simulink model "flight_simulation_6dof"  (R2025b)
settings: Solver=ode4  StartTime=0.0  StopTime=8.6  FixedStep=1/1000  RelTol=1e-3  AbsTol=1e-3  EnableMultiTasking=on
undefined symbols (not defined in the file): X, Y, Z
libraries: nesl_utility x122, sm_lib x98, simulink_extras x48, aerolibatmos2 x4, sharedtransform x4
(part 2 of 6)

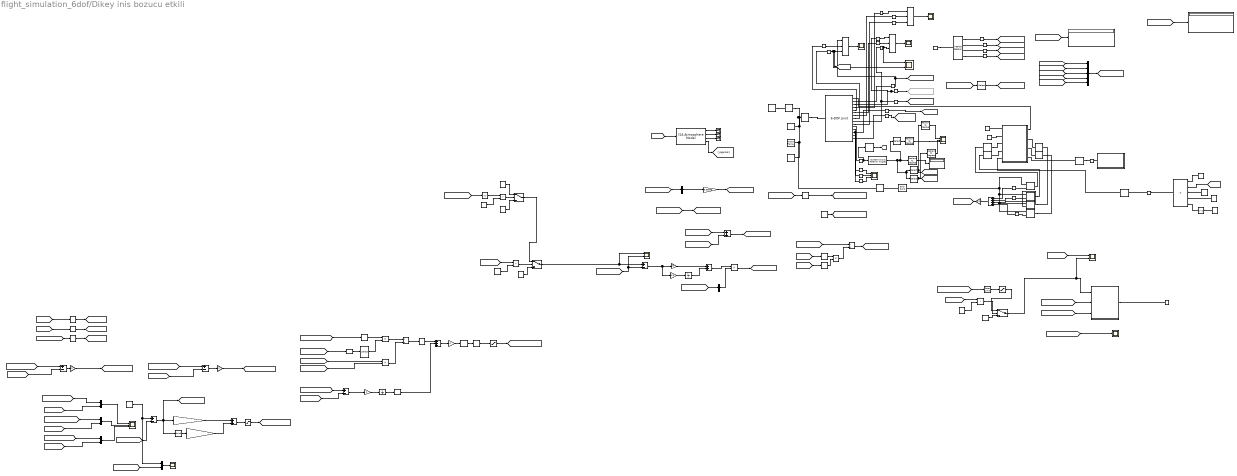
== system flight_simulation_6dof/Dikey inis bozucu etkili ==
  note: 0 itki [N]
  note: Integral Corrector
  note: Ang Velocity to Ang Accel Command
  note: Dynamic Inversion
  note: Ang Velocity to Ang Accel Command
  note: Z Axis
  note: zemine 0.001 metre kala itkiyi 0 yap
  note: Yere 6 metre kala
  note: 6. metreden sonra hizi su olcak
  note: F=1/2 ​ρ.C D. ​A.V rel ​^2
  6-DOF Joint : sm_lib/Joints/6-DOF Joint  JointMode=Normal  CompositeWrenchDir=FollowerOnBase  CompositeWrenchFrame=BaseFrame  SenseConstraintForce=off  SenseConstraintTorque=off  SenseTotalForce=off  SenseTotalTorque=off  PxPositionTargetSpecify=off  PxPositionTargetPriority=High  PxPositionTargetValue=15  PxPositionTargetValueUnits=m  PxVelocityTargetSpecify=off  PxVelocityTargetPriority=High  PxVelocityTargetValue=0  PxVelocityTargetValueUnits=m/s  PxEquilibriumPosition=0  PxEquilibriumPositionUnits=m  PxSpringStiffness=0  PxSpringStiffnessUnits=N/m  PxDampingCoefficient=0  PxDampingCoefficientUnits=N/(m/s)  PxLowerLimitSpecify=off  PxLowerLimitBound=-1  PxLowerLimitBoundUnits=m  PxLowerLimitStiffness=1e6  PxLowerLimitStiffnessUnits=N/m  PxLowerLimitDamping=1e3  PxLowerLimitDampingUnits=N/(m/s)  PxLowerLimitTransitionRegionWidth=1e-4  PxLowerLimitTransitionRegionWidthUnits=m  PxUpperLimitSpecify=off  PxUpperLimitBound=1  PxUpperLimitBoundUnits=m  PxUpperLimitStiffness=1e6  PxUpperLimitStiffnessUnits=N/m  PxUpperLimitDamping=1e3  PxUpperLimitDampingUnits=N/(m/s)  PxUpperLimitTransitionRegionWidth=1e-4  PxUpperLimitTransitionRegionWidthUnits=m  PxTorqueActuationMode=NoTorque  PxMotionActuationMode=ComputedMotion  PxSensePosition=on  PxSenseVelocity=on  PxSenseAcceleration=on  PxSenseTorqueForce=off  PxSenseLowerLimitTorqueForce=off  PxSenseUpperLimitTorqueForce=off  PyPositionTargetSpecify=on  PyPositionTargetPriority=High  PyPositionTargetValue=0  PyPositionTargetValueUnits=m  PyVelocityTargetSpecify=off  PyVelocityTargetPriority=High  PyVelocityTargetValue=0  PyVelocityTargetValueUnits=m/s  PyEquilibriumPosition=0  PyEquilibriumPositionUnits=m  PySpringStiffness=0  PySpringStiffnessUnits=N/m  PyDampingCoefficient=0  PyDampingCoefficientUnits=N/(m/s)  PyLowerLimitSpecify=off  PyLowerLimitBound=-1  PyLowerLimitBoundUnits=m  PyLowerLimitStiffness=1e6  PyLowerLimitStiffnessUnits=N/m  PyLowerLimitDamping=1e3  PyLowerLimitDampingUnits=N/(m/s)  PyLowerLimitTransitionRegionWidth=1e-4  PyLowerLimitTransitionRegionWidthUnits=m  PyUpperLimitSpecify=off  PyUpperLimitBound=1  PyUpperLimitBoundUnits=m  PyUpperLimitStiffness=1e6  PyUpperLimitStiffnessUnits=N/m  PyUpperLimitDamping=1e3  PyUpperLimitDampingUnits=N/(m/s)  PyUpperLimitTransitionRegionWidth=1e-4  PyUpperLimitTransitionRegionWidthUnits=m  PyTorqueActuationMode=NoTorque  PyMotionActuationMode=ComputedMotion  PySensePosition=on  PySenseVelocity=on  PySenseAcceleration=on  PySenseTorqueForce=off  PySenseLowerLimitTorqueForce=off  PySenseUpperLimitTorqueForce=off  PzPositionTargetSpecify=on  PzPositionTargetPriority=High  PzPositionTargetValue=10  PzPositionTargetValueUnits=m  PzVelocityTargetSpecify=off  PzVelocityTargetPriority=High  PzVelocityTargetValue=0  PzVelocityTargetValueUnits=m/s  PzEquilibriumPosition=0  PzEquilibriumPositionUnits=m  PzSpringStiffness=0  PzSpringStiffnessUnits=N/m  PzDampingCoefficient=0  PzDampingCoefficientUnits=N/(m/s)  PzLowerLimitSpecify=off  PzLowerLimitBound=-1  PzLowerLimitBoundUnits=m  PzLowerLimitStiffness=1e6  PzLowerLimitStiffnessUnits=N/m  PzLowerLimitDamping=1e3  PzLowerLimitDampingUnits=N/(m/s)  PzLowerLimitTransitionRegionWidth=1e-4  PzLowerLimitTransitionRegionWidthUnits=m  PzUpperLimitSpecify=off  PzUpperLimitBound=1  PzUpperLimitBoundUnits=m  PzUpperLimitStiffness=1e6  PzUpperLimitStiffnessUnits=N/m  PzUpperLimitDamping=1e3  PzUpperLimitDampingUnits=N/(m/s)  PzUpperLimitTransitionRegionWidth=1e-4  PzUpperLimitTransitionRegionWidthUnits=m  PzTorqueActuationMode=NoTorque  PzMotionActuationMode=ComputedMotion  PzSensePosition=on  PzSenseVelocity=on  PzSenseAcceleration=on  PzSenseTorqueForce=off  PzSenseLowerLimitTorqueForce=off  PzSenseUpperLimitTorqueForce=off  SphPositionTargetSpecify=on  SphPositionTargetPriority=High  SphPositionTargetRotationMethod=StandardAxis  SphPositionTargetFollAlignAxisA=+X  SphPositionTargetBaseAlignAxisA=+Y  SphPositionTargetFollAlignAxisB=+Y  SphPositionTargetBaseAlignAxisB=+Z  SphPositionTargetRotationStandardAxis=+Y  SphPositionTargetRotationAngle=15  SphPositionTargetRotationAngleUnits=deg  SphPositionTargetRotationArbitraryAxis=[1 1 0]  SphPositionTargetRotationSequenceAxes=FollowerAxes  SphPositionTargetRotationSequence=XYX  SphPositionTargetRotationSequenceAngles=[0 0 0]  SphPositionTargetRotationSequenceAnglesUnits=deg  SphPositionTargetRotationMatrix=[1 0 0;0 1 0;0 0 1]  SphPositionTargetQuaternion=[1 0 0 0]  SphVelocityTargetSpecify=off  SphVelocityTargetPriority=High  SphVelocityTargetValue=[0 0 0]  SphVelocityTargetValueUnits=deg/s  SphVelocityTargetInFollowerFrame=on  SphEqPosRotationMethod=None  SphEqPosFollAlignAxisA=+X  SphEqPosBaseAlignAxisA=+Y  SphEqPosFollAlignAxisB=+Y  SphEqPosBaseAlignAxisB=+Z  SphEqPosRotationStandardAxis=+Z  SphEqPosRotationAngle=0  SphEqPosRotationAngleUnits=deg  SphEqPosRotationArbitraryAxis=[0 0 1]  SphEqPosRotationSequenceAxes=FollowerAxes  SphEqPosRotationSequence=XYX  SphEqPosRotationSequenceAngles=[0 0 0]  SphEqPosRotationSequenceAnglesUnits=deg  SphEqPosRotationMatrix=[1 0 0;0 1 0;0 0 1]  SphEqPosQuaternion=[1 0 0 0]  SphSpringStiffness=0  SphSpringStiffnessUnits=N*m/deg  SphDampingCoefficient=0  SphDampingCoefficientUnits=N*m/(deg/s)  SphLowerLimitSpecify=off  SphLowerLimitBound=15  SphLowerLimitBoundUnits=deg  SphLowerLimitStiffness=1e4  SphLowerLimitStiffnessUnits=N*m/deg  SphLowerLimitDamping=10  SphLowerLimitDampingUnits=N*m/(deg/s)  SphLowerLimitTransitionRegionWidth=0.1  SphLowerLimitTransitionRegionWidthUnits=deg  SphUpperLimitSpecify=off  SphUpperLimitBound=45  SphUpperLimitBoundUnits=deg  SphUpperLimitStiffness=1e4  SphUpperLimitStiffnessUnits=N*m/deg  SphUpperLimitDamping=10  SphUpperLimitDampingUnits=N*m/(deg/s)  SphUpperLimitTransitionRegionWidth=0.1  SphUpperLimitTransitionRegionWidthUnits=deg  SphTorqueActuationMode=NoTorque  SphActuateTorqueX=off  SphActuateTorqueY=off  SphActuateTorqueZ=off  SphActuateTorque=off  SphActuationFrame=BaseFrame  SphSensePosition=on  SphSenseVelocityX=on  SphSenseVelocityY=on  SphSenseVelocityZ=on  SphSenseVelocity=off  SphSenseAccelerationX=off  SphSenseAccelerationY=on  SphSenseAccelerationZ=off  SphSenseAcceleration=off  SphSenseLowerLimitTorqueMag=off  SphSenseUpperLimitTorqueMag=off  SphSensingFrame=BaseFrame
  Abs : Abs  SaturateOnIntegerOverflow=off
  Add : Sum
  Add{1..3,5..6} (5 alike) : Sum  Inputs=+-
  Add4 : Sum  Inputs=3
  Add7 : Sum
  Add8 : Sum  Inputs=4
  Add9 : Sum
  Alan : Constant  Value=0.25
  Asin1 : Trigonometry  Operator=asin
  Bus Creator : BusCreator  Inputs=5
  Bus Selector : BusSelector  OutputSignals=mass_kg
  Bus Selector1 : BusSelector  OutputSignals=mass_kg
  CD​≈1 : Constant
  Connection Label16 : ConnectionLabel  Label=FN1
  Connection Label17 : ConnectionLabel  Label=FN1
  Connection Label34 : ConnectionLabel  Label=Nozzle_Frame
  Connection Label35 : ConnectionLabel  Label=Nozzle_Frame
  Constant : Constant  Value=0
  Constant1 : Constant
  Constant2 : Constant  Value=6
  Constant4 : Constant  Value=1/2
  Constant5 : Constant  Value=0
  Constant6 : Constant  Value=-0.08
  Constant7 : Constant  Value=0.001
  Constant8 : Constant  Value=0
  Cos : Trigonometry  Operator=cos
  Cos1 : Trigonometry  Operator=cos
  Degrees to Radians1 : simulink_extras/Transformations/Degrees to Radians
  Degrees to Radians2 : simulink_extras/Transformations/Degrees to Radians
  Delay : Delay  DelayLength=1
  Delay1 : Delay  DelayLength=1  InitialCondition=25000*10
  Derivative : Derivative
  Display : Display
  Display1 : Display
  Display2 : Display
  Divide : Product  Inputs=*/
  Divide2 : Product  Inputs=*/
  External Force and Torque : sm_lib/Forces and Torques/External Force and Torque  EnableForceX=on  EnableForceY=off  EnableForceZ=off  EnableForce=off  ForceResolutionFrame=AttachedFrame  EnableTorqueX=off  EnableTorqueY=off  EnableTorqueZ=off  EnableTorque=off  TorqueResolutionFrame=AttachedFrame
  Floor : sm_lib/Body Elements/Brick Solid  BrickDimensions=[30 30 2]  BrickDimensionsUnits=m  ExportEntireGeometry=on  InertiaType=CalculateFromGeometry  BasedOnType=Density  Density=0  DensityUnits=kg/m^3  Mass=1  MassUnits=kg  CenterOfMass=[0 0 0]  CenterOfMassUnits=m  MomentsOfInertia=[1 1 1]  MomentsOfInertiaUnits=kg*m^2  ProductsOfInertia=[0 0 0]  ProductsOfInertiaUnits=kg*m^2  GraphicType=FromGeometry  MarkerShape=Sphere  MarkerSize=10  GraphicVisPropType=SimpleVisualProperties  GraphicDiffuseColor=[0.4 0.8 0.0]  GraphicOpacity=1  GraphicSpecularColor=[0.5 0.5 0.5 1.0]  GraphicAmbientColor=[0.15 0.15 0.15 1.0]  GraphicEmissiveColor=[0.0 0.0 0.0 1.0]  GraphicShininess=75  DoExposeReferenceFrame=on  SerializedFrames=<Frames/>
  Gain : Gain  Gain=9.80665
  Gain1 : Gain  Gain=1/4
  Gain2 : Gain  Gain=3
  Gain3 : Gain  Gain=0.263030697386858*5
  Gain4 : Gain
  Gain5 : Gain  Gain=2
  Gain6 : Gain  Gain=-1
  Gain7 : Gain  Gain=2
  Gain8 : Gain  Gain=1.772424617277137*2
  Gain9 : Gain  Gain=0.5
  Goto26 : Goto  Commented=on  GotoTag=x_dot_current_m_s
  Graphic : sm_lib/Body Elements/Graphic  GraphicType=Marker  MarkerShape=Cube  MarkerSize=10  GraphicVisPropType=SimpleVisualProperties  GraphicDiffuseColor=[0.5 0.5 0.5]  GraphicOpacity=1  GraphicSpecularColor=[0.5 0.5 0.5 1.0]  GraphicAmbientColor=[0.15 0.15 0.15 1.0]  GraphicEmissiveColor=[0.0 0.0 0.0 1.0]  GraphicShininess=75
  GreaterThan : RelationalOperator  Operator=>  OutDataTypeStr=boolean  RndMeth=Simplest  InputSameDT=off
  GreaterThan1 : RelationalOperator  Operator=>  OutDataTypeStr=boolean  RndMeth=Simplest  InputSameDT=off
  GreaterThan3 : RelationalOperator  Operator=>  OutDataTypeStr=boolean  RndMeth=Simplest  InputSameDT=off
  ISA Atmosphere Model : aerolibatmos2/ISA Atmosphere Model  useExtended=off  action=None  custom=off  viscosityOut=off  g=9.80665  gamma=1.4  R=287.0531  L=0.0065  h_trop=11000  h_strat=20000  rho0=1.225  P0=101325  T0=288.15  h0=0  S=110.4  Tref=273.15  muref=1.716e-5
  Inertia Sensor : sm_lib/Body Elements/Inertia Sensor  SensorExtent=Mechanism  SpanWeldJoints=off  ExcludeGroundedBodies=off  MeasurementFrame=Attached  SenseMass=on  SenseCenterOfMass=on  SenseInertiaMatrix=on  SenseCenteredInertiaMatrix=on  SensePrincipalInertiaMatrix=off  SenseRotationMatrix=off  GraphicType=PrincipalInertiaFrame  PrincipalInertiaFrameSize=20  GraphicVisPropType=SimpleVisualProperties  GraphicDiffuseColor=[0.5 0.5 0.5]  GraphicOpacity=1  GraphicSpecularColor=[0.5 0.5 0.5 1.0]  GraphicAmbientColor=[0.15 0.15 0.15 1.0]  GraphicEmissiveColor=[0.0 0.0 0.0 1.0]  GraphicShininess=75
  Integrator : Integrator  LimitOutput=on  UpperSaturationLimit=10  LowerSaturationLimit=-10
  Integrator1 : Integrator  LimitOutput=on  UpperSaturationLimit=5000*10  LowerSaturationLimit=-5000*10
  MassModel1 : Subsystem
  Mechanism Configuration : sm_lib/Utilities/Mechanism Configuration  UniformGravity=Constant  GravityVector=[0 0 -9.80665]  GravityVectorUnits=m/s^2  LinearizationDelta=0.001  JointModeTransitionNonlinearIterations=2
  Mux{,1..3} (4 alike) : Mux  Inputs=2
  Mux4 : Mux  Inputs=3
  Mux5 : Mux  Inputs=3
  Mux6 : Mux  Inputs=3
  PS-Simulink Converter{,1..24} (25 alike) : nesl_utility/PS-Simulink Converter  PhysicalDomain=network_engine_domain  SubClassName=ps_output  LeftPortType=input  RightPortType=output  PseudoPeriodic=off  Frequencies=[]  VectorFormat=inherit  Unit=inherit  AffineConversion=off
  Product{,1,4..5} (4 alike) : Product
  Product2 : Product  Inputs=5
  Quaternions to Direction Cosine Matrix : Quat2Dcm
  Quaternions to Rotation Angles : sharedtransform/Quaternions to Rotation Angles  rotationOrder=ZYX  aMode=aMode
  Radians to Degrees{,1..4,7..9} (8 alike) : simulink_extras/Transformations/Radians to Degrees
  Rate Limiter : RateLimiter  RisingSlewLimit=500/0.2  FallingSlewLimit=-500/0.2  SampleTimeMode=inherited
  Reshape1 : Reshape
  Rigid Transform : sm_lib/Frames and Transforms/Rigid Transform  RotationMethod=None  FollAlignAxisA=+X  BaseAlignAxisA=+Y  FollAlignAxisB=+Y  BaseAlignAxisB=+Z  RotationStandardAxis=+Z  RotationAngle=0  RotationAngleUnits=deg  RotationArbitraryAxis=[0 0 1]  RotationSequenceAxes=FollowerAxes  RotationSequence=XYX  RotationSequenceAngles=[0 0 0]  RotationSequenceAnglesUnits=deg  RotationMatrix=[1 0 0;0 1 0;0 0 1]  Quaternion=[1 0 0 0]  TranslationMethod=Cartesian  TranslationCartesianOffset=[0 0 0]  TranslationCartesianOffsetUnits=m  TranslationStandardAxis=+Z  TranslationStandardOffset=0  TranslationStandardOffsetUnits=m  TranslationROffset=0  TranslationROffsetUnits=m  TranslationThetaOffset=0  TranslationThetaOffsetUnits=deg  TranslationZOffset=0  TranslationZOffsetUnits=m
  Rigid Transform1 : sm_lib/Frames and Transforms/Rigid Transform  RotationMethod=None  FollAlignAxisA=+X  BaseAlignAxisA=+Y  FollAlignAxisB=+Y  BaseAlignAxisB=+Z  RotationStandardAxis=+Z  RotationAngle=0  RotationAngleUnits=deg  RotationArbitraryAxis=[0 0 1]  RotationSequenceAxes=FollowerAxes  RotationSequence=XYX  RotationSequenceAngles=[0 0 0]  RotationSequenceAnglesUnits=deg  RotationMatrix=[1 0 0;0 1 0;0 0 1]  Quaternion=[1 0 0 0]  TranslationMethod=Cartesian  TranslationCartesianOffset=[0 0 -1.82]  TranslationCartesianOffsetUnits=m  TranslationStandardAxis=+Z  TranslationStandardOffset=0  TranslationStandardOffsetUnits=m  TranslationROffset=0  TranslationROffsetUnits=m  TranslationThetaOffset=0  TranslationThetaOffsetUnits=deg  TranslationZOffset=0  TranslationZOffsetUnits=m
  Rigid Transform2 : sm_lib/Frames and Transforms/Rigid Transform  RotationMethod=None  FollAlignAxisA=+X  BaseAlignAxisA=+Y  FollAlignAxisB=+Y  BaseAlignAxisB=+Z  RotationStandardAxis=+Z  RotationAngle=0  RotationAngleUnits=deg  RotationArbitraryAxis=[0 0 1]  RotationSequenceAxes=FollowerAxes  RotationSequence=XYX  RotationSequenceAngles=[0 0 0]  RotationSequenceAnglesUnits=deg  RotationMatrix=[1 0 0;0 1 0;0 0 1]  Quaternion=[1 0 0 0]  TranslationMethod=Cartesian  TranslationCartesianOffset=[0 0 -1.82]  TranslationCartesianOffsetUnits=m  TranslationStandardAxis=+Z  TranslationStandardOffset=0  TranslationStandardOffsetUnits=m  TranslationROffset=0  TranslationROffsetUnits=m  TranslationThetaOffset=0  TranslationThetaOffsetUnits=deg  TranslationZOffset=0  TranslationZOffsetUnits=m
  Saturation : Saturate  UpperLimit=60  LowerLimit=-60
  Saturation1 : Saturate  UpperLimit=20  LowerLimit=-20
  Saturation2 : Saturate  UpperLimit=500/0.2  LowerLimit=0
  Scope : Scope  NumInputPorts=2
      settings: ActiveDisplayYMinimum=-1.625829118727711  ActiveDisplayYMaximum=0.25053784432938375
  Scope1 : Scope  NumInputPorts=3
      settings: ActiveDisplayYMinimum=-19.808742904399047  ActiveDisplayYMaximum=34.576797333379531
  Scope10 : Scope  NumInputPorts=2
      settings: ActiveDisplayYMinimum=-107.28824489550837  ActiveDisplayYMaximum=965.56718541932582  DataLoggingVariableName=ScopeData9
  Scope11 : Scope  NumInputPorts=3
      settings: ActiveDisplayYMinimum=-22.793707101323157  ActiveDisplayYMaximum=10.917952452796278  DataLoggingVariableName=ScopeData12
  Scope{2,5..7,9} (5 alike) : Scope
      Scope2 settings: ActiveDisplayYMinimum=-1  ActiveDisplayYMaximum=1  DataLoggingVariableName=ScopeData2
      Scope5 settings: ActiveDisplayYMinimum=-11.092753948931176  ActiveDisplayYMaximum=5.4980270582822843  DataLoggingVariableName=ScopeData3
      Scope6 settings: ActiveDisplayYMinimum=-2.6747294131347727  ActiveDisplayYMaximum=11.408303268126085  DataLoggingVariableName=ScopeData4
      Scope7 settings: ActiveDisplayYMinimum=-50.120004759868806  ActiveDisplayYMaximum=49.994550495676052  DataLoggingVariableName=ScopeData5
      Scope9 settings: ActiveDisplayYMinimum=-1  ActiveDisplayYMaximum=1  DataLoggingVariableName=ScopeData8
  Scope4 : Scope  NumInputPorts=2
      settings: ActiveDisplayYMinimum=-9.5328876838367336  ActiveDisplayYMaximum=0.53135333799624407  DataLoggingVariableName=ScopeData7
  Scope8 : Scope  NumInputPorts=3
      settings: ActiveDisplayYMinimum=-25.077488901630971  ActiveDisplayYMaximum=26.517066183158931  DataLoggingVariableName=ScopeData10
  Selector : Selector  InputPortWidth=3  IndexOptions=Index vector (dialog)  Indices=2  OutputSizes=1
  Selector1 : Selector  InputPortWidth=3  IndexOptions=Index vector (dialog)  Indices=3  OutputSizes=1
  Selector2 : Selector  InputPortWidth=3  IndexOptions=Index vector (dialog)  Indices=3  OutputSizes=1
  Selector3 : Selector  InputPortWidth=3  IndexOptions=Index vector (dialog)  Indices=1  OutputSizes=1
  Selector4 : Selector  InputPortWidth=9  IndexOptions=Index vector (dialog)  Indices=5  OutputSizes=1
  Simulink-PS Converter : nesl_utility/Simulink-PS Converter  PhysicalDomain=network_engine_domain  SubClassName=ps_input  LeftPortType=input  RightPortType=output  PseudoPeriodic=off  Frequencies=[]  NoiseDistribution=none  NoiseParameters=[]  Unit=1  AffineConversion=off  FilteringAndDerivatives=provide  SimscapeFilterOrder=1  InputFilterTimeConstant=0.001  UdotUserProvided=0
  Simulink-PS Converter2 : nesl_utility/Simulink-PS Converter  PhysicalDomain=network_engine_domain  SubClassName=ps_input  LeftPortType=input  RightPortType=output  PseudoPeriodic=off  Frequencies=[]  NoiseDistribution=none  NoiseParameters=[]  Unit=1  AffineConversion=off  FilteringAndDerivatives=provide  SimscapeFilterOrder=1  InputFilterTimeConstant=0.001  UdotUserProvided=0
  Solver Configuration : nesl_utility/Solver Configuration  PhysicalDomain=network_engine_domain  SubClassName=solver  LeftPortType=input  RightPortType=generic  Tones=[]  Harmonics=[]  SimulateNoise=off  Profile=off  UseLocalSampling=off  EnableSwitchedLinearOptims=on  FrequencyDomain=off  UseCCode=off  RelTol=0.001  AbsTol=1e-06  MinStep=1e-09  ToWorkspace=off  RevertToSquareIcSolve=off  NumHomotopyIterations=100  PhasorMode=off  PhasorModeNumHarmonics=1  ConsistencySolver=NEWTON_XTOL_AFTER_FTOL  IndexReductionMethod=DerivativeReplacement  DoDC=off  ResidualTolerance=1e-09  ConsistencyTolSource=GLOBAL  ConsistencyAbsTol=0.001  ConsistencyRelTol=0.001  ConsistencyTolFactor=0.001  UseLocalSolver=off  LocalSolverChoice=NE_BACKWARD_EULER_ADVANCER  ResolveIndetEquations=on  FunctionEvalNumThread=1  LocalSolverSampleTime=0.001  DoFixedCost=off  MaxNonlinIter=3  MaxModeIter=2  ComputeImpulses=off  ImpulseIterations=2  LinearAlgebra=Sparse  LinearAlgebraNumThread=0  EquationFormulation=NE_TIME_EF  DelaysMemoryBudget=1024  AutomaticFiltering=on  FilteringTimeConstant=0.001  PartitionStorageMethod=AS_NEEDED  PartitionMemoryBudget=1024  PartitionMethod=FAST  MultibodyUseLocalSolver=off  MultibodyLocalSolverChoice=ODE1  MultibodyLocalSolverSampleTime=0.001
  Spatial Contact Force{,1..3} (4 alike) : sm_lib/Forces and Torques/Spatial Contact Force  SenseSeparationDistance=on  NormalForceType=SmoothSpringDamper  NormalStiffness=3e4  NormalStiffnessUnits=N/m  NormalDamping=8e2  NormalDampingUnits=N/(m/s)  NormalTransitionRegionWidth=1e-3  NormalTransitionRegionWidthUnits=m  FrictionType=SmoothStickSlip  CoefficientOfStaticFriction=0.5  CoefficientOfDynamicFriction=0.3  FrictionalCriticalVelocity=1e-3  FrictionalCriticalVelocityUnits=m/s  SenseContactSignal=off  SensePenetrationDepth=off  SenseNormalVelocity=off  SenseTangentialVelocity=off  SensingForceTorqueDirection=BaseOnFollower  SensingForceTorqueResolutionFrame=ContactFrame  SenseNormalForce=off  SenseNormalForceMagnitude=off  SenseNormalTorque=off  SenseFrictionalForce=off  SenseFrictionalForceMagnitude=off  SenseFrictionalTorque=off  SenseTotalForce=off  SenseTotalTorque=off  SenseContactBaseRotation=off  SenseContactBaseTranslation=off  SenseContactFollowerRotation=off  SenseContactFollowerTranslation=off  ZeroCrossDetectContactStartAndEnd=off
  Spherical Solid{,1..3} (4 alike) : sm_lib/Body Elements/Spherical Solid  SphereRadius=0.01  SphereRadiusUnits=m  ExportEntireGeometry=on  InertiaType=CalculateFromGeometry  BasedOnType=Density  Density=0  DensityUnits=kg/m^3  Mass=1  MassUnits=kg  CenterOfMass=[0 0 0]  CenterOfMassUnits=m  MomentsOfInertia=[1 1 1]  MomentsOfInertiaUnits=kg*m^2  ProductsOfInertia=[0 0 0]  ProductsOfInertiaUnits=kg*m^2  GraphicType=FromGeometry  MarkerShape=Sphere  MarkerSize=10  GraphicVisPropType=SimpleVisualProperties  GraphicDiffuseColor=[0.502 0 0]  GraphicOpacity=1  GraphicSpecularColor=[0.5 0.5 0.5 1.0]  GraphicAmbientColor=[0.15 0.15 0.15 1.0]  GraphicEmissiveColor=[0.0 0.0 0.0 1.0]  GraphicShininess=75  DoExposeReferenceFrame=on  SerializedFrames=<Frames/>
  Square : Math  Operator=square
  Subsystem : Subsystem
      mask Display: image('ktr_roket_gorseli.jfif');
  Subsystem2 : Subsystem
      mask Display: image('WhatsApp Image 2026-05-11 at 00.40.18.jpeg');
  Switch : Switch  Criteria=u2 > Threshold  SaturateOnIntegerOverflow=off  InputSameDT=off
  Switch1 : Switch  Criteria=u2 > Threshold  SaturateOnIntegerOverflow=off  InputSameDT=off
  Switch3 : Switch  Criteria=u2 > Threshold  SaturateOnIntegerOverflow=off  InputSameDT=off
  Terminator : Terminator
  Terminator1 : Terminator
  Terminator2 : Terminator
  Variable Cylindrical Solid : sm_lib/Body Elements/Variable Mass/Variable Cylindrical Solid  RadiusType=Constant  Radius=0.1  RadiusUnits=m  LengthType=Constant  Length=0.4002  LengthUnits=m  MassType=ProvidedByInput  Density=1000  DensityUnits=kg/m^3  SenseRadius=off  SenseLength=off  SenseMass=off  SenseCenterOfMass=off  SenseInertiaMatrix=off  GraphicType=FromGeometry  MarkerShape=Sphere  MarkerSize=10  GraphicVisPropType=SimpleVisualProperties  GraphicDiffuseColor=[0.5 0.5 0.5]  GraphicOpacity=1  GraphicSpecularColor=[0.5 0.5 0.5 1.0]  GraphicAmbientColor=[0.15 0.15 0.15 1.0]  GraphicEmissiveColor=[0.0 0.0 0.0 1.0]  GraphicShininess=75
  Vrel​ : Constant  Value=6
  World Frame : sm_lib/Frames and Transforms/World Frame
  X Command [m] : Constant  Value=0
  itki devreye girene kadar serbest dusus hizi : Constant  Value=-10.85
  wires:
  Quaternions to Direction Cosine Matrix/1 -> [DCM]
  ISA Atmosphere Model/4 -> [yogunluk]  "Yogunluk"
  ISA Atmosphere Model/2 -> Terminator1/1
  ISA Atmosphere Model/3 -> Terminator2/1
  ISA Atmosphere Model/1 -> Terminator/1
  [z_current_m] -> ISA Atmosphere Model/1  "Z Konumu"
  Switch3/1 -> Subsystem2/1(Thrust Commanded[N]), Scope10/2  "itki N"
  Saturation2/1 -> Switch3/1  "Thrust_Comannded"
  [Thrust_Commanded_N] -> Rate Limiter/1
  Constant8/1 -> Switch3/3
  [Ground_Distance_m] -> GreaterThan3/1
  Constant7/1 -> GreaterThan3/2
  GreaterThan3/1 -> Switch3/2
  Switch1/1 -> Add1/1, Scope/1  "Vz_Command"
  PS-Simulink Converter24/1 -> Scope11/3  "r"
  PS-Simulink Converter23/1 -> Scope11/2  "q"
  PS-Simulink Converter22/1 -> Scope11/1  "p"
  Radians to Degrees9/1 -> Scope8/3  "Roll"
  Selector3/1 -> Radians to Degrees9/1
  Radians to Degrees8/1 -> Scope8/2  "Pitch"
  Radians to Degrees7/1 -> Scope8/1  "Yaw"
  [Ground_Distance_m] -> Scope10/1  "Ground_distance"
  Rate Limiter/1 -> Saturation2/1
  Constant6/1 -> Switch1/3
  Switch/1 -> Switch1/1  "Vz_Command"
  GreaterThan1/1 -> Switch1/2
  [Ground_Distance_m] -> GreaterThan1/1
  Constant2/1 -> GreaterThan1/2
  Gain1/1 -> [Ground_Distance_m]
  Add8/1 -> Gain1/1
  PS-Simulink Converter1/1 -> Add8/1
  PS-Simulink Converter19/1 -> Add8/2
  PS-Simulink Converter20/1 -> Add8/3
  PS-Simulink Converter21/1 -> Add8/4
  MassModel1/1(Mass of Gas [kg]) -> Simulink-PS Converter/1  "m(t)"
  PS-Simulink Converter18/1 -> [mass_kg]
  [theta_rad] -> Radians to Degrees1/1
  [Frame_Angle_1_Commanded_deg] -> Scope9/1
  itki devreye girene kadar serbest dusus hizi/1 -> Switch/3
  Constant5/1 -> Switch/1
  GreaterThan/1 -> Switch/2
  Constant1/1 -> GreaterThan/2
  Abs/1 -> GreaterThan/1
  [error_x_m] -> Abs/1
  [Frame_Angle_2_Commanded_deg] -> Subsystem2/3(Frame Angle 2 Commanded[°])
  [Frame_Angle_1_Commanded_deg] -> Subsystem2/2(Frame Angle Commanded[°])
  [CG_m] -> Display2/1  "CG_m"
  Mux6/1 -> Scope7/1
  PS-Simulink Converter17/1 -> Mux6/3  "Z Ekseni İvme"
  PS-Simulink Converter16/1 -> Mux6/2  "Y Ekseni İvme"
  PS-Simulink Converter15/1 -> Mux6/1  "X Ekseni İvme"
  Mux5/1 -> Scope5/1
  PS-Simulink Converter14/1 -> Mux5/3, Scope4/1  "Z Ekseni Hız"
  PS-Simulink Converter13/1 -> Mux5/2  "Y Ekseni Hız"
  PS-Simulink Converter12/1 -> Mux5/1  "X Ekseni Hız"
  PS-Simulink Converter10/1 -> Mux4/3, [z_current_m], Scope4/2  "Z Ekseni Konumu"
  PS-Simulink Converter11/1 -> Mux4/2  "Y Ekseni Konumu"
  Mux4/1 -> Scope6/1
  Add9/1 -> Product/1
  Integrator1/1 -> Add9/2
  Gain9/1 -> Integrator1/1
  Add7/1 -> Saturation1/1
  Gain8/1 -> Add7/2
  Derivative/1 -> Gain8/1
  PS-Simulink Converter9/1 -> Goto26/1
  [x_current_m] -> Mux3/2
  Mux3/1 -> Scope2/1
  X Command [m]/1 -> Add6/1, Mux3/1  "X Command [m]"
  Saturation1/1 -> [ang_command_deg]
  Gain3/1 -> Add7/1
  [x_current_m] -> Add6/2
  PS-Simulink Converter8/1 -> [x_current_m], Mux4/1  "X Ekseni Konumu"
  Radians to Degrees4/1 -> [ang_accel_deg_s2]
  Radians to Degrees2/1 -> [ang_vel_deg_s]
  Radians to Degrees1/1 -> [angle_deg]
  [theta_dot_dot_rad_s2] -> Radians to Degrees4/1
  [theta_dot_rad_s] -> Radians to Degrees2/1
  PS-Simulink Converter7/1 -> [theta_dot_dot_rad_s2]
  PS-Simulink Converter6/1 -> [theta_dot_rad_s]
  Gain5/1 -> [ang_accel_Command_deg_s2]  "angular_accel_command_deg"
  [ang_command_deg] -> Mux2/1  "angle_command_deg"
  [ang_accel_deg_s2] -> Mux/2
  Mux2/1 -> Scope1/1  "Pos"
  Product4/1 -> Divide2/1
  Radians to Degrees3/1 -> Saturation/1
  Degrees to Radians2/1 -> Add4/2
  [ang_vel_command_deg_s] -> Mux1/1
  Mux/1 -> Scope1/3  "Accel"
  Selector4/1 -> Product4/2
  [ang_accel_deg_s2] -> Add3/2
  [angle_deg] -> Mux2/2  "angle_deg"
  Reshape1/1 -> Selector4/1
  Product5/1 -> Divide2/2
  Asin1/1 -> Add4/1
  [ang_accel_Command_deg_s2] -> Mux/1
  Integrator/1 -> Degrees to Radians2/1
  Gain4/1 -> Integrator/1
  Delay/1 -> Radians to Degrees3/1
  Add3/1 -> Gain4/1
  [ang_accel_Command_deg_s2] -> Degrees to Radians1/1
  Add6/1 -> Gain3/1, [error_x_m], Derivative/1
  Add2/1 -> Gain5/1
  Add4/1 -> Gain6/1
  Divide2/1 -> Asin1/1
  [ang_vel_deg_s] -> Add2/2
  [ang_accel_Command_deg_s2] -> Add3/1
  Mux1/1 -> Scope1/2  "Vel"
  [ang_vel_command_deg_s] -> Add2/1  "angular_velocity_command_deg"
  [FT_N] -> Product5/2
  [ang_vel_deg_s] -> Mux1/2
  Add5/1 -> Gain7/1
  Saturation/1 -> [Frame_Angle_1_Commanded_deg]
  Gain7/1 -> [ang_vel_command_deg_s]  "ang_vel_command_deg_s"
  [ang_command_deg] -> Add5/1  "angular_velocity_command_deg"
  [moment_arm_m] -> Product5/1
  Gain6/1 -> Delay/1
  [angle_deg] -> Add5/2
  [centered_inertia_kgm2] -> Reshape1/1
  Degrees to Radians1/1 -> Product4/1
  Selector2/1 -> [moment_arm_m]
  Selector/1 -> Radians to Degrees7/1, [theta_rad]
  Add1/1 -> Gain2/1, Gain9/1
  Bus Selector1/1 -> Product/2  "<mass_kg>"
  [Delta_FT] -> Add/2
  [Vz_Current_m_s] -> Scope/2, Add1/2  "Vz_Current"
  [FT_N] -> Delay1/1
  PS-Simulink Converter2/1 -> [CG_m]
  Gain/1 -> [FG_N]
  Delay1/1 -> [Thrust_Commanded_N]
  Divide/1 -> [FT_N]
  Product1/1 -> Divide/2
  Add/1 -> [FT_Z_N]
  PS-Simulink Converter4/1 -> Quaternions to Rotation Angles/1, Quaternions to Direction Cosine Matrix/1
  Cos/1 -> Product1/1
  PS-Simulink Converter/1 -> [Vz_Current_m_s]
  Product/1 -> [Delta_FT]
  [CG_m] -> Selector2/1
  [CG_m] -> Bus Creator/2  "CG_m"
  [theta_rad] -> Cos/1
  Constant/1 -> [Frame_Angle_2_Commanded_deg]
  [inertia_kgm2] -> Bus Creator/3  "inertia_kgm2"
  Bus Creator/1 -> [inertial_parameters]
  Bus Selector/1 -> Gain/1  "<mass_kg>"
  PS-Simulink Converter3/1 -> [inertia_kgm2]
  [phi_rad] -> Cos1/1
  [mass_kg] -> Bus Creator/1  "mass_kg"
  Radians to Degrees/1 -> Display/1
  Cos1/1 -> Product1/2
  [inertial_parameters] -> Bus Selector1/1
  [inertial_parameters] -> Bus Selector/1
  Selector1/1 -> [phi_rad], Radians to Degrees8/1
  [FG_N] -> [FT_0]
  [centered_inertia_kgm2] -> Bus Creator/5  "centered_inertia_kgm2"
  [centered_inertia_kgm2] -> Display1/1
  Gain2/1 -> Add9/1
  [moment_arm_m] -> Bus Creator/4  "moment_arm_m"
  [FT_0] -> Add/1
  [FT_Z_N] -> Divide/1
  PS-Simulink Converter5/1 -> [centered_inertia_kgm2]
  Quaternions to Rotation Angles/1 -> Radians to Degrees/1, Selector3/1, Selector/1, Selector1/1
  Constant4/1 -> Product2/1
  Square/1 -> Product2/5
  Alan/1 -> Product2/4
  Product2/1 -> Simulink-PS Converter2/1
  CD​≈1/1 -> Product2/3
  Vrel​/1 -> Square/1
  [yogunluk] -> Product2/2
  connections:
  Rigid Transform/LConn1 -- Solver Configuration/RConn1 -- Mechanism Configuration/RConn1 -- Rigid Transform1/LConn1 -- World Frame/RConn1 -- Rigid Transform2/LConn1
  Floor/RConn1 -- Rigid Transform1/RConn1
  6-DOF Joint/RConn14 -- PS-Simulink Converter24/LConn1
  6-DOF Joint/RConn12 -- PS-Simulink Converter22/LConn1
  Spatial Contact Force3/RConn2 -- PS-Simulink Converter21/LConn1
  Spatial Contact Force2/RConn2 -- PS-Simulink Converter20/LConn1
  Spatial Contact Force1/RConn2 -- PS-Simulink Converter19/LConn1
  Spatial Contact Force/RConn2 -- PS-Simulink Converter1/LConn1
  Spatial Contact Force3/LConn1 -- Spherical Solid3/LConn1
  Spatial Contact Force2/LConn1 -- Spherical Solid2/LConn1
  Spatial Contact Force1/LConn1 -- Spherical Solid1/LConn1
  Variable Cylindrical Solid/LConn1 -- Simulink-PS Converter/RConn1
  Inertia Sensor/RConn1 -- PS-Simulink Converter18/LConn1
  Spatial Contact Force/LConn1 -- Spherical Solid/LConn1
  6-DOF Joint/RConn10 -- PS-Simulink Converter17/LConn1
  6-DOF Joint/RConn7 -- PS-Simulink Converter16/LConn1
  6-DOF Joint/RConn4 -- PS-Simulink Converter15/LConn1
  6-DOF Joint/RConn6 -- PS-Simulink Converter13/LConn1
  6-DOF Joint/RConn5 -- PS-Simulink Converter11/LConn1
  6-DOF Joint/RConn8 -- PS-Simulink Converter10/LConn1
  Spatial Contact Force2/RConn1 -- Spatial Contact Force3/RConn1 -- Spatial Contact Force1/RConn1 -- Floor/LConn1 -- Spatial Contact Force/RConn1
  PS-Simulink Converter9/LConn1 -- PS-Simulink Converter12/LConn1 -- 6-DOF Joint/RConn3
  PS-Simulink Converter8/LConn1 -- 6-DOF Joint/RConn2
  PS-Simulink Converter7/LConn1 -- 6-DOF Joint/RConn15
  6-DOF Joint/RConn13 -- PS-Simulink Converter23/LConn1 -- PS-Simulink Converter6/LConn1
  Inertia Sensor/RConn4 -- PS-Simulink Converter5/LConn1
  PS-Simulink Converter4/LConn1 -- 6-DOF Joint/RConn11
  PS-Simulink Converter3/LConn1 -- Inertia Sensor/RConn3
  Rigid Transform/RConn1 -- 6-DOF Joint/LConn1
  PS-Simulink Converter14/LConn1 -- 6-DOF Joint/RConn9 -- PS-Simulink Converter/LConn1
  Subsystem2/RConn1 -- Connection Label17/LConn1
  PS-Simulink Converter2/LConn1 -- Inertia Sensor/RConn2
  Connection Label35/LConn1 -- Inertia Sensor/LConn1
  Graphic/RConn1 -- Rigid Transform2/RConn1
  Subsystem/RConn1 -- 6-DOF Joint/RConn1
  Subsystem/LConn1 -- Connection Label34/LConn1
  Subsystem/LConn2 -- Connection Label16/LConn1
  Spherical Solid/RConn1 -- Subsystem/LConn3
  Spherical Solid2/RConn1 -- Subsystem/RConn2
  Subsystem/LConn4 -- Spherical Solid1/RConn1
  Spherical Solid3/RConn1 -- Subsystem/RConn3
  Variable Cylindrical Solid/RConn1 -- Subsystem/RConn4
  External Force and Torque/RConn1 -- Subsystem/LConn5
  Simulink-PS Converter2/RConn1 -- External Force and Torque/LConn1
